simulink model "commhdlQPSKTxRx"  (R2025b)
settings: Solver=FixedStepDiscrete  StartTime=0.0  StopTime=stopTime  RelTol=1e-3
PostLoadFcn:
  | hScopeConfig = get_param([gcs '/Receiver/QPSK Rx/Frequency and Time Synchronizer/Symbol Synchronizer/No HDL/QPSK Receiver Eye Diagram'],'ScopeConfiguration');
  | 
  | hScopeConfig.OpenAtSimulationStart = false;
  | hScopeConfig.Visible = false;
  | SamplesPerSymbol = 4;
  | %UpsamplesRx = 1;
  | clear hScopeConfig
InitFcn:
  | commhdlQPSKTxRxModelInit;
  | % Rate bridge: ADRV9002/Jupiter radio runs at 15.36 MHz = 2x the 7.68 MHz
  | % (4 samples/symbol @ Rsym=1.92 MHz) the QPSK Rx requires. The deployed
  | % Receiver must downsample the ADC stream by 2. UpsamplesRx=1 fed the QPSK
  | % Rx 8 sps (2x-upsampled) and broke symbol sync / the loopback bit check.
  | UpsamplesRx = 1;   %% T8 RATE FIX: rail 15.36e6 == ADC bus rate,
  | %% no ingress decimation (was 2 when the rail sat on the 7.68e6 rung)
  | UpsamplesTx = 1;
  | clear simTimingOffset;
StopFcn:
  | if exist('simTimingOffset','var')
  |   disp('Simulation completed');
  |   %QPSKTxRxVerification;
  | end
undefined symbols (not defined in the file or in its folder): Add, Config, fsym, randsrc, RandStream, Rsym, Shift
libraries: hdlsllib x76, simulink x21, dspsigops x19, dsphdlfiltering2 x3, dsphdlsigops2 x2, dsphdlmathfun2 x2, commdigbbndpm3 x2, commchan3 x1, commrflib2 x1
(part 2 of 4)

== system commhdlQPSKTxRx/Transmitter/QPSK Tx/HDL Data Scrambler ==
  note: HDL Data Scrambler
      | Polynomial: x^7+x^4+1
      | Initial state: [1 0 1 1 1 0 1]
  dataIn : Inport
  startIn : Inport  Port=2
  endIn : Inport  Port=3
  validIn : Inport  Port=4
  BIT_XOR : Logic  Operator=XOR  IconShape=distinctive  AllPortsSameDT=off  OutDataTypeStr=boolean
  BIT_XOR2 : Logic  Operator=XOR  IconShape=distinctive  AllPortsSameDT=off  OutDataTypeStr=boolean
  Delay{,1,3..4} (4 alike) : Delay  DelayLength=1
  EnableScrambling : Constant  Value=true  SampleTime=-1
  Logical Operator : Logic  IconShape=distinctive  AllPortsSameDT=off  OutDataTypeStr=boolean
  Switch : Switch  Criteria=u2 > Threshold  SaturateOnIntegerOverflow=off  InputSameDT=off
  Unit Delay Enabled Resettable Synchronous{,2..3,5,7} (5 alike) : hdlsllib/Discrete/Unit Delay Enabled Resettable Synchronous  InitialCondition=1  SampleTime=-1
  Unit Delay Enabled Resettable Synchronous1 : hdlsllib/Discrete/Unit Delay Enabled Resettable Synchronous  InitialCondition=0  SampleTime=-1
  Unit Delay Enabled Resettable Synchronous4 : hdlsllib/Discrete/Unit Delay Enabled Resettable Synchronous  InitialCondition=0  SampleTime=-1
  Unit Delay Enabled Resettable Synchronous6 : hdlsllib/Discrete/Unit Delay Enabled Resettable Synchronous  InitialCondition=0.0  SampleTime=-1
  dataOut : Outport  InitialOutput=0
  validOut : Outport  Port=2  InitialOutput=0
  wires:
  Delay4/1 -> validOut/1
  Delay3/1 -> dataOut/1
  endIn/1 -> Unit Delay Enabled Resettable Synchronous4/3
  Logical Operator/1 -> BIT_XOR2/2
  Unit Delay Enabled Resettable Synchronous4/1 -> Logical Operator/1
  Delay1/1 -> Unit Delay Enabled Resettable Synchronous6/2, Unit Delay Enabled Resettable Synchronous2/2, Unit Delay Enabled Resettable Synchronous1/2, Unit Delay Enabled Resettable Synchronous/2, Delay4/1, Unit Delay Enabled Resettable Synchronous3/2, Unit Delay Enabled Resettable Synchronous5/2, Unit Delay Enabled Resettable Synchronous7/2
  Delay/1 -> Switch/3, BIT_XOR2/1
  startIn/1 -> Unit Delay Enabled Resettable Synchronous4/1, Unit Delay Enabled Resettable Synchronous4/2, Unit Delay Enabled Resettable Synchronous6/3, Unit Delay Enabled Resettable Synchronous5/3, Unit Delay Enabled Resettable Synchronous1/3, Unit Delay Enabled Resettable Synchronous/3, Unit Delay Enabled Resettable Synchronous2/3, Unit Delay Enabled Resettable Synchronous3/3, Unit Delay Enabled Resettable Synchronous7/3
  dataIn/1 -> Delay/1
  validIn/1 -> Delay1/1
  BIT_XOR/1 -> Unit Delay Enabled Resettable Synchronous/1, Logical Operator/2
  Unit Delay Enabled Resettable Synchronous1/1 -> Unit Delay Enabled Resettable Synchronous2/1
  Unit Delay Enabled Resettable Synchronous2/1 -> Unit Delay Enabled Resettable Synchronous3/1
  Unit Delay Enabled Resettable Synchronous/1 -> Unit Delay Enabled Resettable Synchronous1/1
  Unit Delay Enabled Resettable Synchronous3/1 -> BIT_XOR/2, Unit Delay Enabled Resettable Synchronous5/1
  Unit Delay Enabled Resettable Synchronous5/1 -> Unit Delay Enabled Resettable Synchronous6/1
  Unit Delay Enabled Resettable Synchronous6/1 -> Unit Delay Enabled Resettable Synchronous7/1
  Unit Delay Enabled Resettable Synchronous7/1 -> BIT_XOR/1
  Switch/1 -> Delay3/1
  EnableScrambling/1 -> Switch/2
  BIT_XOR2/1 -> Switch/1

== system commhdlQPSKTxRx/Transmitter/QPSK Tx/QPSK Modulator ==
  dataIn : Inport
  validIn : Inport  Port=2
  Compare To Constant : simulink/Logic and Bit Operations/Compare To Constant  relop===  const=0  OutDataTypeStr=boolean
  Compare To Constant1 : simulink/Logic and Bit Operations/Compare To Constant  relop===  const=1  OutDataTypeStr=boolean
  Delay{,1..5,11..12} (8 alike) : Delay  DelayLength=1
  HDL Counter : hdlsllib/Sources/HDL Counter  CountType=Count limited  CountInit=0  CountStep=1  CountMax=1  CountFromType=Initial value  CountFrom=0  CountResetPort=off  CountLoadPort=off  CountEnbPort=on  CountDirPort=off  CountHitOutputPort=off  CountDataType=Unsigned  CountWordLen=1  CountFracLen=0  CountSampTime=1
  Logical Operator : Logic  IconShape=distinctive  AllPortsSameDT=off  OutDataTypeStr=boolean
  Logical Operator1 : Logic  IconShape=distinctive  AllPortsSameDT=off  OutDataTypeStr=boolean
  Mux : Mux  Inputs=2
  Null : Constant  Value=complex(0,0)  OutDataTypeStr=fixdt(1,16,15)  SampleTime=1/(Rsym*SamplesPerSymbol)
  QPSK Modulator Baseband : commdigbbndpm3/QPSK Modulator Baseband  InType=Bit  Enc=Gray  Ph=pi/4  outDtype=Fixed-point  outWordLen=16  outUDDataType=sfix(16)  outFracLenMode=User-defined  outFracLen=15  outDataTypeStr=fixdt(1,16,15)  outLastDataTypeStr=fixdt(1,16,15)
  Switch3 : Switch  Threshold=1  SaturateOnIntegerOverflow=off  InputSameDT=off
  Unit Delay Enabled Synchronous : hdlsllib/Discrete/Unit Delay Enabled Synchronous  InitialCondition=0.0  SampleTime=-1
  dataOut : Outport
  validOut : Outport  Port=2
  wires:
  dataIn/1 -> Delay/1
  validIn/1 -> Delay1/1
  HDL Counter/1 -> Compare To Constant/1, Compare To Constant1/1
  QPSK Modulator Baseband/1 -> Delay11/1
  Logical Operator1/1 -> Delay5/1
  Switch3/1 -> Delay2/1
  Null/1 -> Switch3/3
  Delay/1 -> Mux/2, Unit Delay Enabled Synchronous/1
  Delay2/1 -> dataOut/1
  Delay3/1 -> validOut/1
  Delay1/1 -> Logical Operator1/2, Logical Operator/1, HDL Counter/1
  Compare To Constant/1 -> Logical Operator/2
  Compare To Constant1/1 -> Logical Operator1/1
  Delay11/1 -> Switch3/1
  Delay12/1 -> Switch3/2, Delay3/1
  Logical Operator/1 -> Unit Delay Enabled Synchronous/2
  Unit Delay Enabled Synchronous/1 -> Mux/1
  Mux/1 -> Delay4/1
  Delay4/1 -> QPSK Modulator Baseband/1
  Delay5/1 -> Delay12/1

== system commhdlQPSKTxRx/Transmitter/QPSK Tx/RRC Transmit Filter ==
  dataIn : Inport
  validIn : Inport  Port=2
  Data Type Conversion : DataTypeConversion  OutDataTypeStr=fixdt(1,17,16)  SaturateOnIntegerOverflow=off  RndMeth=Floor
  Data Type Conversion1 : DataTypeConversion  OutDataTypeStr=fixdt(1,16,14)  SaturateOnIntegerOverflow=off  RndMeth=Floor
  Delay1 : Delay  DelayLength=1
  Delay2 : Delay  DelayLength=1
  Delay3 : Delay  DelayLength=1
  RRC Filter : dsphdlfiltering2/Discrete FIR Filter  NumeratorSource=Property  Numerator=RRCCoef  NumeratorPrototype=[]  FilterStructure=Direct form systolic  SerializationOption=Minimum number of cycles between valid input samples  NumCycles=2  NumberOfMultipliers=2  SimulateUsing=Code generation  roundingMode=Floor  overflowMode=off  CoefficientsDataTypeStr=Inherit: Same word length as input  OutputDataTypeStr=Inherit: Same word length as input  ResetInputPort=off  HDLGlobalReset=off  CoeffMultiplier=Multiplier  UseMultForPow2Coeff=on  FrameInputSymmOptim=off
  Unit Delay Enabled Synchronous1 : hdlsllib/Discrete/Unit Delay Enabled Synchronous  InitialCondition=0  SampleTime=-1
  dataOut : Outport
  validOut : Outport  Port=2
  wires:
  dataIn/1 -> Data Type Conversion/1
  RRC Filter/1 -> Data Type Conversion1/1
  RRC Filter/2 -> Delay2/1
  Delay1/1 -> dataOut/1
  Delay2/1 -> validOut/1
  Data Type Conversion/1 -> Delay3/1
  Unit Delay Enabled Synchronous1/1 -> RRC Filter/2
  Data Type Conversion1/1 -> Delay1/1
  validIn/1 -> Unit Delay Enabled Synchronous1/2, Unit Delay Enabled Synchronous1/1
  Delay3/1 -> RRC Filter/1

== system commhdlQPSKTxRx/Receiver/QPSK Rx/Automatic Gain Control/Error Detector ==
  dataIn : Inport
  Add1 : Sum  Inputs=+-
  Conj : Math  Operator=conj
  Data Type Duplicate : DataTypeDuplicate
  Delay{,1..3} (4 alike) : Delay
  Product : Product
  Ref : Constant  Value=Ref  OutDataTypeStr=Inherit: Inherit via back propagation  SampleTime=-1
  err : Outport
  wires:
  Delay3/1 -> err/1
  Delay2/1 -> Add1/2
  Delay1/1 -> Product/1
  Delay/1 -> Product/2
  Ref/1 -> Data Type Duplicate/1, Add1/1
  Conj/1 -> Delay/1
  Product/1 -> Delay2/1
  dataIn/1 -> Conj/1, Data Type Duplicate/2, Delay1/1
  Add1/1 -> Delay3/1

== system commhdlQPSKTxRx/Receiver/QPSK Rx/Automatic Gain Control/Loop Filter ==
  note: Fixed point precision loss warnings
      | are supressed in Mask Init Callback
  err : Inport
  Add : Sum  Inputs=|++  OutDataTypeStr=Inherit: Same as first input
  Delay1 : Delay  DelayLength=1
  Delay2 : Delay
  Delay3 : Delay
  Gain1 : Gain  Gain=LFG  OutDataTypeStr=fixdt(1,34,28)
      mask init:
      | Simulink.suppressDiagnostic(gcb, 'SimulinkFixedPoint:util:fxpParameterPrecisionLoss');
  gain : Outport
  wires:
  Delay3/1 -> Gain1/1
  Delay2/1 -> Add/1
  Gain1/1 -> Delay2/1
  Add/1 -> Delay1/1
  Delay1/1 -> Add/2, gain/1
  err/1 -> Delay3/1

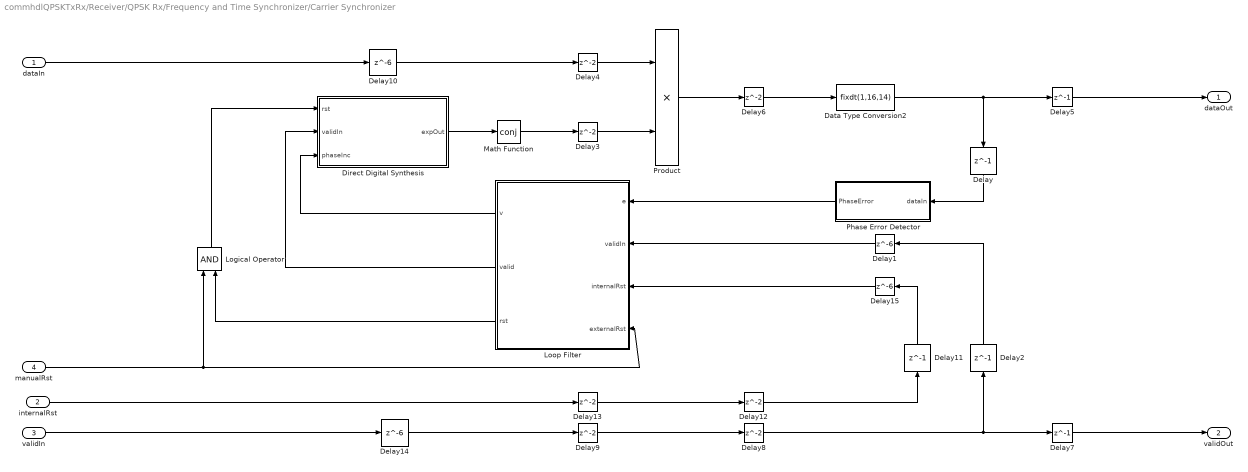
== system commhdlQPSKTxRx/Receiver/QPSK Rx/Frequency and Time Synchronizer/Carrier Synchronizer ==
  dataIn : Inport
  internalRst : Inport  Port=2
  validIn : Inport  Port=3
  manualRst : Inport  Port=4
  Data Type Conversion2 : DataTypeConversion  OutDataTypeStr=fixdt(1,16,14)  SaturateOnIntegerOverflow=off  RndMeth=Floor
  Delay{,2,5,7,11} (5 alike) : Delay  DelayLength=1
  Delay{1,10,14..15} (4 alike) : Delay  DelayLength=6
  Delay{3..4,6,8..9,12..13} (7 alike) : Delay
  Direct Digital Synthesis : Subsystem
  Logical Operator : Logic  AllPortsSameDT=off  OutDataTypeStr=boolean
  Loop Filter : Subsystem
  Math Function : Math  Operator=conj  SignedPower=on  RndMeth=Zero
  Phase Error Detector : Subsystem
  Product : Product
  dataOut : Outport
  validOut : Outport  Port=2
  wires:
  Delay/1 -> Phase Error Detector/1(dataIn)
  Math Function/1 -> Delay3/1
  Data Type Conversion2/1 -> Delay5/1, Delay/1
  Delay3/1 -> Product/2
  Product/1 -> Delay6/1
  Delay8/1 -> Delay2/1, Delay7/1
  Delay9/1 -> Delay8/1
  Delay4/1 -> Product/1
  Delay6/1 -> Data Type Conversion2/1
  Direct Digital Synthesis/1(expOut) -> Math Function/1
  Loop Filter/1(v) -> Direct Digital Synthesis/3(phaseInc)
  Phase Error Detector/1(PhaseError) -> Loop Filter/1(e)
  Delay2/1 -> Delay1/1
  Delay1/1 -> Loop Filter/2(validIn)
  Delay10/1 -> Delay4/1
  Delay11/1 -> Delay15/1
  Delay12/1 -> Delay11/1
  Delay13/1 -> Delay12/1
  Loop Filter/2(valid) -> Direct Digital Synthesis/2(validIn)
  Delay5/1 -> dataOut/1
  Delay7/1 -> validOut/1
  dataIn/1 -> Delay10/1
  internalRst/1 -> Delay13/1
  validIn/1 -> Delay14/1
  Delay14/1 -> Delay9/1
  manualRst/1 -> Logical Operator/1, Loop Filter/4(externalRst)
  Delay15/1 -> Loop Filter/3(internalRst)
  Loop Filter/3(rst) -> Logical Operator/2
  Logical Operator/1 -> Direct Digital Synthesis/1(rst)

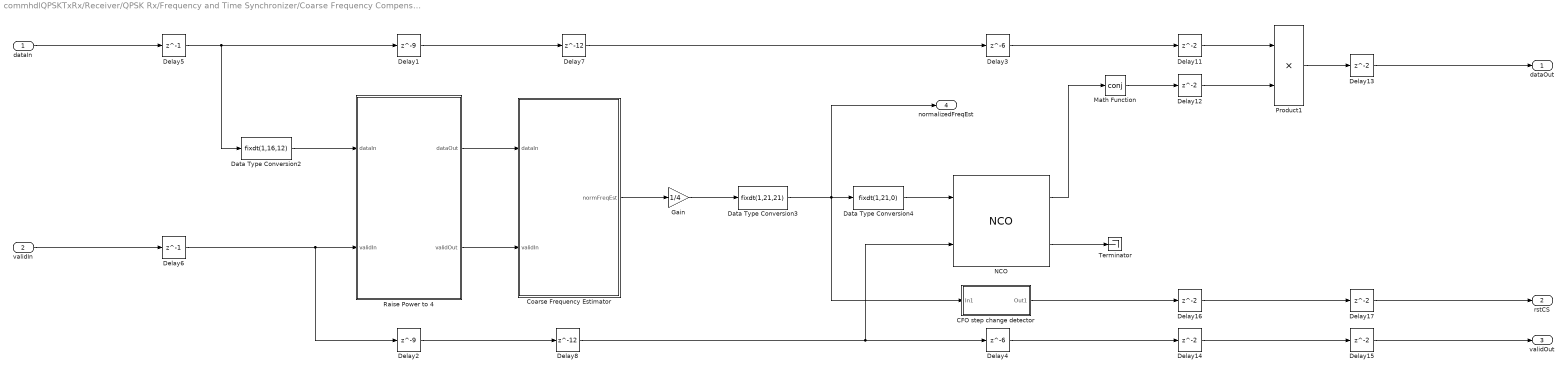
== system commhdlQPSKTxRx/Receiver/QPSK Rx/Frequency and Time Synchronizer/Coarse Frequency Compensator ==
  dataIn : Inport
  validIn : Inport  Port=2
  CFO step change detector : Subsystem
  Coarse Frequency Estimator : Subsystem
  Data Type Conversion2 : DataTypeConversion  OutDataTypeStr=fixdt(1,16,12)  SaturateOnIntegerOverflow=off  RndMeth=Floor
  Data Type Conversion3 : DataTypeConversion  OutDataTypeStr=fixdt(1,21,21)  SaturateOnIntegerOverflow=off  RndMeth=Floor
  Data Type Conversion4 : DataTypeConversion  OutDataTypeStr=fixdt(1,21,0)  ConvertRealWorld=Stored Integer (SI)  SaturateOnIntegerOverflow=off  RndMeth=Floor
  Delay1 : Delay  DelayLength=9
  Delay{11..17} (7 alike) : Delay
  Delay2 : Delay  DelayLength=9
  Delay3 : Delay  DelayLength=6
  Delay4 : Delay  DelayLength=6
  Delay5 : Delay  DelayLength=1
  Delay6 : Delay  DelayLength=1
  Delay7 : Delay  DelayLength=12
  Delay8 : Delay  DelayLength=12
  Gain : Gain  Gain=1/4  ParamDataTypeStr=fixdt(0,2,2)  OutDataTypeStr=Inherit: Same as input
  Math Function : Math  Operator=conj
  NCO : dsphdlsigops2/NCO  PhaseIncrementSource=Input port  PhaseIncrement=100  PhaseOffsetSource=Property  PhaseOffset=0  DitherSource=None  NumDitherBits=4  SamplesPerFrame=1  LUTCompress=off  ResetAction=off  Waveform=Complex exponential  PhasePort=off  SimulateUsing=Code generation  AccumulatorWL=21  PhaseQuantization=on  NumQuantizerAccumulatorBits=14  OutputDataType=Binary point scaling  OutputWL=16  OutputFL=14
  Product1 : Product  OutDataTypeStr=Inherit: Same as first input
  Raise Power to 4 : Subsystem
  Terminator : Terminator
  dataOut : Outport
  rstCS : Outport  Port=2
  validOut : Outport  Port=3
  normalizedFreqEst : Outport  Port=4
  wires:
  Delay14/1 -> Delay15/1
  Delay11/1 -> Product1/1
  Delay6/1 -> Raise Power to 4/2(validIn), Delay2/1
  Delay5/1 -> Delay1/1, Data Type Conversion2/1
  Data Type Conversion4/1 -> NCO/1
  Delay4/1 -> Delay14/1
  Delay3/1 -> Delay11/1
  Delay2/1 -> Delay8/1
  Delay1/1 -> Delay7/1
  NCO/2 -> Terminator/1
  NCO/1 -> Math Function/1
  Product1/1 -> Delay13/1
  Raise Power to 4/2(validOut) -> Coarse Frequency Estimator/2(validIn)
  Math Function/1 -> Delay12/1
  Raise Power to 4/1(dataOut) -> Coarse Frequency Estimator/1(dataIn)
  Delay12/1 -> Product1/2
  Coarse Frequency Estimator/1(normFreqEst) -> Gain/1
  Data Type Conversion2/1 -> Raise Power to 4/1(dataIn)
  Delay16/1 -> Delay17/1
  CFO step change detector/1(Out1) -> Delay16/1
  Gain/1 -> Data Type Conversion3/1
  Delay13/1 -> dataOut/1
  dataIn/1 -> Delay5/1
  validIn/1 -> Delay6/1
  Delay17/1 -> rstCS/1
  Data Type Conversion3/1 -> normalizedFreqEst/1, CFO step change detector/1(In1), Data Type Conversion4/1
  Delay15/1 -> validOut/1
  Delay7/1 -> Delay3/1
  Delay8/1 -> NCO/2, Delay4/1

== system commhdlQPSKTxRx/Receiver/QPSK Rx/Frequency and Time Synchronizer/No HDL ==
  In1 : Inport
  In2 : Inport  Port=2
  In3 : Inport  Port=3
  In4 : Inport  Port=4
  Data Type Conversion : DataTypeConversion  OutDataTypeStr=double  SaturateOnIntegerOverflow=off  RndMeth=Floor
  Data Type Conversion1 : DataTypeConversion  OutDataTypeStr=double  SaturateOnIntegerOverflow=off  RndMeth=Floor
  QPSK Receiver Constellations 2 : ConstellationDiagram  NumInputPorts=2  WindowPosition=[67.000000,180.000000,973.000000,678.000000,]  Visible=on  ScopeFrameLocation=window  SymbolsToDisplaySource=Property  SymbolsToDisplay=10000  ReferenceConstellation="{[0.70711+0.70711i        -0.70711+0.70711i        -0.70711-0.70711i         0.70711-0.70711i],[0.70711+0.70711i        -0.70711+0.70711i        -0.70711-0.70711i         0.70711-0.70711i]}"  ReferenceMarker={''+'',''+''}  ReferenceColor={[1 0 0],[1 0 0]}  XLimits=[-1.3581 1.3569]  YLimits=[-1.3581 1.3569]  AxesLimits=[-1.3581 1.3569]  ShowLegend=on  DefaultConfigurationName=comm.scopes.ConstellationDiagramBlockCfg
      settings: OpenAtSimulationStart=off
  Subsystem : Subsystem
  Unit Delay Enabled Synchronous : hdlsllib/Discrete/Unit Delay Enabled Synchronous  InitialCondition=0.0  SampleTime=-1
  Unit Delay Enabled Synchronous1 : hdlsllib/Discrete/Unit Delay Enabled Synchronous  InitialCondition=0.0  SampleTime=-1
  wires:
  In4/1 -> Unit Delay Enabled Synchronous1/2, Subsystem/Enable
  Data Type Conversion/1 -> Unit Delay Enabled Synchronous1/1, Subsystem/1(In1)
  Unit Delay Enabled Synchronous1/1 -> QPSK Receiver Constellations 2/2  "After Carrier Synchronization"
  In2/1 -> Unit Delay Enabled Synchronous/2
  In1/1 -> Data Type Conversion1/1
  Data Type Conversion1/1 -> Unit Delay Enabled Synchronous/1
  Unit Delay Enabled Synchronous/1 -> QPSK Receiver Constellations 2/1  "After Symbol Synchronization"
  In3/1 -> Data Type Conversion/1

== system commhdlQPSKTxRx/Receiver/QPSK Rx/Frequency and Time Synchronizer/Packet Controller ==
  dataIn : Inport
  syncPulse : Inport  Port=2
  validIn : Inport  Port=3
  Delay : Delay  DelayLength=4
  Delay1 : Delay  DelayLength=4
  Delay2 : Delay  DelayLength=4
  End Generator : Subsystem
  Logical Operator : Logic  IconShape=distinctive  AllPortsSameDT=off  OutDataTypeStr=boolean
  MATLAB Function : MATLAB Function  TreatAsAtomicUnit=on
  Time Scope End Generator : Scope  Commented=on  NumInputPorts=2
      settings: SampleTime=1  ActiveDisplayYMinimum=-0.048155737704917989  ActiveDisplayYMaximum=1.0464480874316939  YLabel=Amplitude  DataLoggingVariableName=ScopeData2
  To File : ToFile  Filename=end_gen.mat  MatrixName=end_gen  SaveFormat=Timeseries
  To File1 : ToFile  Filename=reset  MatrixName=reset  SaveFormat=Timeseries
  sample discard controller : MATLAB Function  TreatAsAtomicUnit=on
  dataOut : Outport
  startOut : Outport  Port=2
  endOut : Outport  Port=3
  validOut : Outport  Port=4
  wires:
  MATLAB Function/1(out) -> Logical Operator/2
  sample discard controller/1(dataOut) -> dataOut/1
  sample discard controller/2(startOut) -> startOut/1
  sample discard controller/3(endOut) -> endOut/1
  sample discard controller/4(validOut) -> validOut/1
  Delay/1 -> sample discard controller/1(dataIn)
  Delay1/1 -> sample discard controller/2(validIn), End Generator/1(validIn)
  Delay2/1 -> sample discard controller/3(startIn)
  dataIn/1 -> Delay/1
  validIn/1 -> MATLAB Function/1(valid), Delay1/1, Logical Operator/1
  Logical Operator/1 -> Delay2/1, To File1/1, Time Scope End Generator/2, End Generator/2(rst)
  syncPulse/1 -> MATLAB Function/2(syncPulse)
  End Generator/1(endOut) -> Time Scope End Generator/1, To File/1, sample discard controller/4(endIn)

== system commhdlQPSKTxRx/Receiver/QPSK Rx/Frequency and Time Synchronizer/Phase Ambiguity Estimation and Correction ==
  dataIn : Inport
  syncPulseIn : Inport  Port=2
  validIn : Inport  Port=3
  Average Estimates : Subsystem
  Delay : Delay  DelayLength=32
  Delay1 : Delay  DelayLength=32
  Delay10 : Delay  DelayLength=15 + 7
  Delay11 : Delay  DelayLength=5
  Delay12 : Delay  DelayLength=5
  Delay13 : Delay  DelayLength=5
  Delay2 : Delay  DelayLength=32
  Delay3 : Delay  DelayLength=8
  Delay4 : Delay  DelayLength=8
  Delay5 : Delay  DelayLength=8
  Delay6 : Delay  DelayLength=1
  Delay7 : Delay  DelayLength=1
  Delay8 : Delay  DelayLength=1
  Delay9 : Delay  DelayLength=10
  Phase Ambiguity Corrector : Subsystem
  Phase Ambiguity Estimator : Subsystem
  dataOut : Outport
  syncPulseOut : Outport  Port=2
  validOut : Outport  Port=3
  wires:
  Delay4/1 -> Delay2/1
  Delay5/1 -> Delay/1
  Delay3/1 -> Delay1/1
  Delay10/1 -> Delay9/1
  Phase Ambiguity Corrector/1(dataOut) -> dataOut/1
  Phase Ambiguity Corrector/2(validOut) -> validOut/1
  Delay9/1 -> syncPulseOut/1
  Delay8/1 -> Phase Ambiguity Corrector/1(dataIn)
  Average Estimates/1(avgEst) -> Phase Ambiguity Corrector/2(estimate)
  Delay7/1 -> Phase Ambiguity Corrector/3(validIn)
  Delay6/1 -> Delay10/1
  dataIn/1 -> Delay5/1
  validIn/1 -> Delay4/1
  Delay13/1 -> Delay8/1
  Phase Ambiguity Estimator/1(endOut) -> Average Estimates/1(endIn)
  Phase Ambiguity Estimator/3(validOut) -> Average Estimates/3(validIn)
  Delay12/1 -> Delay7/1
  Delay11/1 -> Delay6/1
  Phase Ambiguity Estimator/2(estOut) -> Average Estimates/2(estin)
  Delay/1 -> Delay13/1, Phase Ambiguity Estimator/1(dataIn)
  syncPulseIn/1 -> Phase Ambiguity Estimator/2(syncPulse), Delay3/1
  Delay2/1 -> Phase Ambiguity Estimator/3(validIn), Delay12/1
  Delay1/1 -> Delay11/1

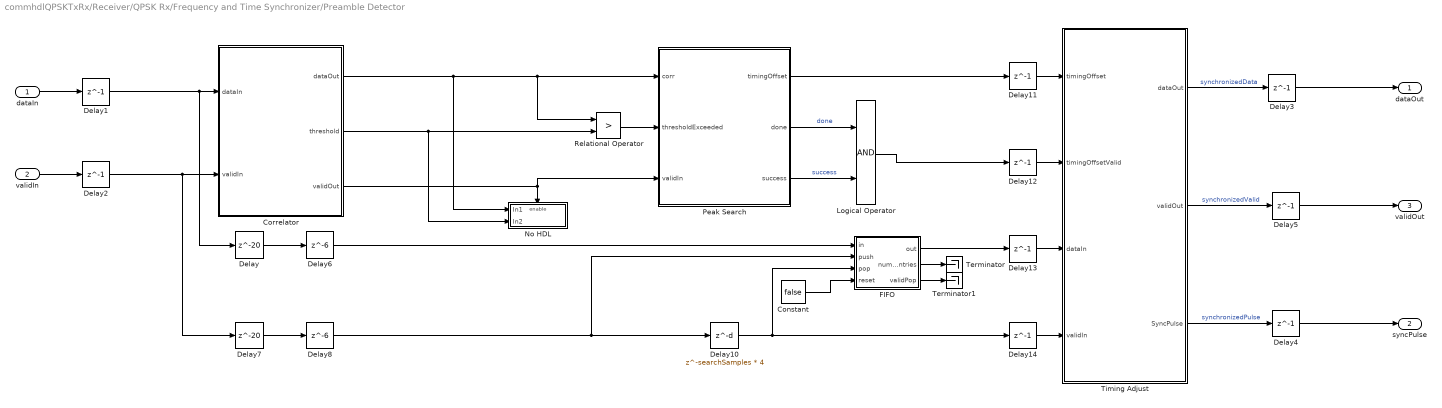
== system commhdlQPSKTxRx/Receiver/QPSK Rx/Frequency and Time Synchronizer/Preamble Detector ==
  dataIn : Inport
  validIn : Inport  Port=2
  Constant : Constant  Value=false  SampleTime=-1
  Correlator : Subsystem
  Delay : Delay  DelayLength=20
  Delay{1..5,11..14} (9 alike) : Delay  DelayLength=1
  Delay10 : Delay  DelayLength=searchSamples * 4
  Delay6 : Delay  DelayLength=6
  Delay7 : Delay  DelayLength=20
  Delay8 : Delay  DelayLength=6
  FIFO : Subsystem  mask{fifoSize=searchSamples, pushFullDiag=Error, popEmptyDiag=Error}
      mask prompts: fifoSize "FIFO size:"; pushFullDiag "Push full FIFO:"; popEmptyDiag "Pop empty FIFO:"
      mask TypeOptions pushFullDiag: Ignore | Warning | Error
      mask TypeOptions popEmptyDiag: Ignore | Warning | Error
  Logical Operator : Logic  AllPortsSameDT=off  OutDataTypeStr=boolean
  No HDL : Subsystem
  Peak Search : Subsystem  VariantControl=new  mask{samplesPerFrame=searchSamples}
      mask prompts: samplesPerFrame "Number of samples to search:"
      mask init:
      | samplesPerFrame1x            = samplesPerFrame;
      |     searchDuration               = samplesPerFrame1x;
  Relational Operator : RelationalOperator  Operator=>  OutDataTypeStr=boolean  InputSameDT=off
  Terminator : Terminator
  Terminator1 : Terminator
  Timing Adjust : Subsystem
  dataOut : Outport
  syncPulse : Outport  Port=2
  validOut : Outport  Port=3
  wires:
  Delay/1 -> Delay6/1
  validIn/1 -> Delay2/1
  dataIn/1 -> Delay1/1
  Relational Operator/1 -> Peak Search/2(thresholdExceeded)
  Peak Search/3(success) -> Logical Operator/2  "success"
  Peak Search/2(done) -> Logical Operator/1  "done"
  Delay7/1 -> Delay8/1
  Timing Adjust/1(dataOut) -> Delay3/1  "synchronizedData"
  Timing Adjust/3(SyncPulse) -> Delay4/1  "synchronizedPulse"
  Timing Adjust/2(validOut) -> Delay5/1  "synchronizedValid"
  Delay3/1 -> dataOut/1
  Delay5/1 -> validOut/1
  Delay4/1 -> syncPulse/1
  Peak Search/1(timingOffset) -> Delay11/1
  Logical Operator/1 -> Delay12/1
  Delay10/1 -> FIFO/3(pop), Delay14/1
  Correlator/3(validOut) -> Peak Search/3(validIn), No HDL/Enable
  Correlator/2(threshold) -> Relational Operator/2, No HDL/2(In2)
  Correlator/1(dataOut) -> Relational Operator/1, Peak Search/1(corr), No HDL/1(In1)
  Delay8/1 -> FIFO/2(push), Delay10/1
  Delay1/1 -> Delay/1, Correlator/1(dataIn)
  Delay2/1 -> Delay7/1, Correlator/2(validIn)
  Delay11/1 -> Timing Adjust/1(timingOffset)
  Delay12/1 -> Timing Adjust/2(timingOffsetValid)
  Delay13/1 -> Timing Adjust/3(dataIn)
  Delay14/1 -> Timing Adjust/4(validIn)
  FIFO/2(numEntries) -> Terminator/1
  Constant/1 -> FIFO/4(reset)
  FIFO/3(validPop) -> Terminator1/1
  Delay6/1 -> FIFO/1(in)
  FIFO/1(out) -> Delay13/1

== system commhdlQPSKTxRx/Receiver/QPSK Rx/Frequency and Time Synchronizer/Symbol Synchronizer ==
  dataIn : Inport
  validIn : Inport  Port=2
  Data Type Conversion4 : DataTypeConversion  OutDataTypeStr=fixdt(1,16,14)  SaturateOnIntegerOverflow=off  RndMeth=Floor
  Delay{1..4,6,8..9} (7 alike) : Delay  DelayLength=1
  Delay5 : Delay  DelayLength=12
  Delay7 : Delay  DelayLength=12
  Gardner TED : Subsystem
  Integer Delay{1..4} (4 alike) : Delay  DelayLength=1
  Interpolation Control : MATLAB Function
  Interpolation Filter : Subsystem
  Loop Filter : Subsystem
  No HDL : Subsystem
  Rate Handle : Subsystem
  dataOut : Outport
  validOut : Outport  Port=2
  wires:
  Loop Filter/1(v) -> Delay4/1
  Gardner TED/1(e) -> Delay3/1
  Interpolation Control/2(Underflow) -> Integer Delay3/1
  Integer Delay4/1 -> Interpolation Filter/2(mu)
  dataIn/1 -> No HDL/1(data), Integer Delay1/1
  Integer Delay3/1 -> Delay5/1
  Delay3/1 -> Loop Filter/1(e)
  Delay4/1 -> Interpolation Control/1(Delta)
  Data Type Conversion4/1 -> Rate Handle/1(dataIn)
  Delay1/1 -> Data Type Conversion4/1
  Delay6/1 -> Rate Handle/3(validIn)
  Delay7/1 -> Delay6/1
  validIn/1 -> No HDL/2(valid), Integer Delay2/1
  Rate Handle/2(validOut) -> validOut/1
  Rate Handle/1(dataOut) -> dataOut/1
  Interpolation Filter/1(interpolant) -> Delay8/1, Delay1/1
  Interpolation Control/1(mu) -> Integer Delay4/1
  Delay2/1 -> Rate Handle/2(strobe)
  Delay5/1 -> Delay9/1, Delay2/1
  Integer Delay1/1 -> Interpolation Filter/1(In)
  Integer Delay2/1 -> Delay7/1
  Delay8/1 -> Gardner TED/1(data)
  Delay9/1 -> Gardner TED/2(strobe)

== system commhdlQPSKTxRx/Receiver/QPSK Rx/QPSK Demodulator/Serializer ==
  u : Inport
  In2 : Inport  Port=2
  Delay1 : Delay  DelayLength=1
  Delay4 : Delay  DelayLength=1
  Demux : Demux  Outputs=2
  HDL Counter : hdlsllib/Sources/HDL Counter  CountType=Count limited  CountInit=0  CountStep=1  CountMax=1  CountFromType=Initial value  CountFrom=0  CountResetPort=off  CountLoadPort=off  CountEnbPort=on  CountDirPort=off  CountHitOutputPort=off  CountDataType=Unsigned  CountWordLen=1  CountFracLen=0  CountSampTime=1
  Logical Operator : Logic  Operator=OR  AllPortsSameDT=off  OutDataTypeStr=boolean
  Multiport Switch : MultiPortSwitch  DataPortOrder=Zero-based contiguous  Inputs=2  zeroidx=on  SaturateOnIntegerOverflow=off  InputSameDT=off
  Unit Delay Enabled Synchronous : hdlsllib/Discrete/Unit Delay Enabled Synchronous  InitialCondition=0.0  SampleTime=-1
  Out1 : Outport
  Out2 : Outport  Port=2
  wires:
  Demux/2 -> Multiport Switch/3
  Logical Operator/1 -> Out2/1, HDL Counter/1
  In2/1 -> Unit Delay Enabled Synchronous/2, Delay1/1
  HDL Counter/1 -> Multiport Switch/1
  Delay4/1 -> Logical Operator/2
  u/1 -> Unit Delay Enabled Synchronous/1
  Multiport Switch/1 -> Out1/1
  Demux/1 -> Multiport Switch/2
  Delay1/1 -> Logical Operator/1, Delay4/1
  Unit Delay Enabled Synchronous/1 -> Demux/1

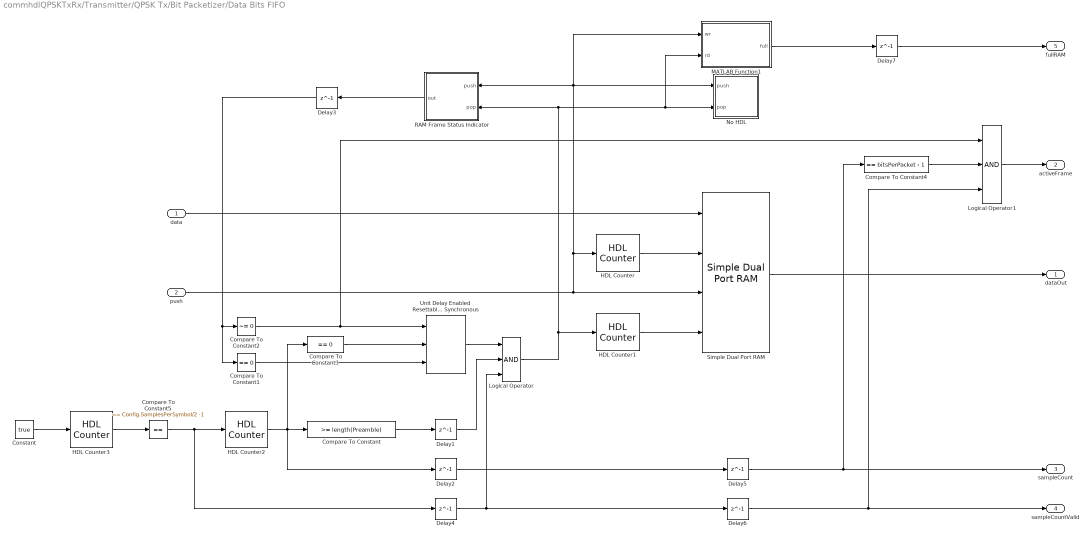
== system commhdlQPSKTxRx/Transmitter/QPSK Tx/Bit Packetizer/Data Bits FIFO ==
  data : Inport
  push : Inport  Port=2
  Compare To Constant : simulink/Logic and Bit Operations/Compare To Constant  relop=>=  const=length(Preamble)  OutDataTypeStr=boolean
  Compare To Constant1 : simulink/Logic and Bit Operations/Compare To Constant  relop===  const=0  OutDataTypeStr=boolean
  Compare To Constant2 : simulink/Logic and Bit Operations/Compare To Constant  relop=~=  const=0  OutDataTypeStr=boolean
  Compare To Constant3 : simulink/Logic and Bit Operations/Compare To Constant  relop===  const=0  OutDataTypeStr=boolean
  Compare To Constant4 : simulink/Logic and Bit Operations/Compare To Constant  relop===  const=bitsPerPacket - 1  OutDataTypeStr=boolean
  Compare To Constant5 : hdlsllib/Logic and Bit Operations/Compare To Constant  relop===  const=Config.SamplesPerSymbol/2 -1  OutDataTypeStr=boolean
  Constant : Constant  Value=true  SampleTime=1/(Rsym*SamplesPerSymbol)
  Delay{1..7} (7 alike) : Delay  DelayLength=1
  HDL Counter : hdlsllib/Sources/HDL Counter  CountType=Count limited  CountInit=0  CountStep=1  CountMax=dataBitsPerPacket*2 - 1  CountFromType=Initial value  CountFrom=0  CountResetPort=off  CountLoadPort=off  CountEnbPort=on  CountDirPort=off  CountHitOutputPort=off  CountDataType=Unsigned  CountWordLen=nextpow2(dataBitsPerPacket*2 - 1)  CountFracLen=0  CountSampTime=1
  HDL Counter1 : hdlsllib/Sources/HDL Counter  CountType=Count limited  CountInit=0  CountStep=1  CountMax=dataBitsPerPacket*2 - 1  CountFromType=Initial value  CountFrom=0  CountResetPort=off  CountLoadPort=off  CountEnbPort=on  CountDirPort=off  CountHitOutputPort=off  CountDataType=Unsigned  CountWordLen=nextpow2(dataBitsPerPacket*2 - 1)  CountFracLen=0  CountSampTime=1
  HDL Counter2 : hdlsllib/Sources/HDL Counter  CountType=Count limited  CountInit=0  CountStep=1  CountMax=bitsPerPacket - 1  CountFromType=Initial value  CountFrom=0  CountResetPort=off  CountLoadPort=off  CountEnbPort=on  CountDirPort=off  CountHitOutputPort=off  CountDataType=Unsigned  CountWordLen=nextpow2(bitsPerPacket)  CountFracLen=0  CountSampTime=1
  HDL Counter3 : hdlsllib/Sources/HDL Counter  CountType=Count limited  CountInit=0  CountStep=1  CountMax=Config.SamplesPerSymbol/2 -1  CountFromType=Initial value  CountFrom=0  CountResetPort=off  CountLoadPort=off  CountEnbPort=on  CountDirPort=off  CountHitOutputPort=off  CountDataType=Unsigned  CountWordLen=nextpow2(Config.SamplesPerSymbol/2)  CountFracLen=0  CountSampTime=1
  Logical Operator : Logic  Inputs=3  AllPortsSameDT=off  OutDataTypeStr=boolean
  Logical Operator1 : Logic  Inputs=3  AllPortsSameDT=off  OutDataTypeStr=boolean
  MATLAB Function1 : MATLAB Function  TreatAsAtomicUnit=on
  No HDL : Subsystem
  RAM Frame Status Indicator : MATLAB Function  TreatAsAtomicUnit=on
  Simple Dual Port RAM : hdlsllib/HDL RAMs/Simple Dual Port RAM  ram_size=nextpow2(dataBitsPerPacket*2 - 1)
  Unit Delay Enabled Resettable Synchronous : hdlsllib/Discrete/Unit Delay Enabled Resettable Synchronous  InitialCondition=0.0  SampleTime=-1
  dataOut : Outport
  activeFrame : Outport  Port=2
  sampleCount : Outport  Port=3
  sampleCountValid : Outport  Port=4
  fullRAM : Outport  Port=5
  wires:
  HDL Counter1/1 -> Simple Dual Port RAM/4
  HDL Counter/1 -> Simple Dual Port RAM/2
  data/1 -> Simple Dual Port RAM/1
  Constant/1 -> HDL Counter3/1
  HDL Counter2/1 -> Compare To Constant/1, Delay2/1, Compare To Constant3/1
  Compare To Constant1/1 -> Unit Delay Enabled Resettable Synchronous/3
  RAM Frame Status Indicator/1(out) -> Delay3/1
  Compare To Constant2/1 -> Logical Operator1/1, Unit Delay Enabled Resettable Synchronous/1
  Compare To Constant3/1 -> Unit Delay Enabled Resettable Synchronous/2
  Compare To Constant/1 -> Delay1/1
  Delay1/1 -> Logical Operator/2
  Delay2/1 -> Delay5/1
  Delay3/1 -> Compare To Constant2/1, Compare To Constant1/1
  Simple Dual Port RAM/1 -> dataOut/1
  Delay4/1 -> Logical Operator/3, Delay6/1
  Delay5/1 -> Compare To Constant4/1, sampleCount/1
  Delay6/1 -> Logical Operator1/3, sampleCountValid/1
  Unit Delay Enabled Resettable Synchronous/1 -> Logical Operator/1
  Compare To Constant4/1 -> Logical Operator1/2
  Logical Operator1/1 -> activeFrame/1
  Logical Operator/1 -> RAM Frame Status Indicator/2(pop), MATLAB Function1/2(rd), No HDL/2(pop), HDL Counter1/1
  push/1 -> MATLAB Function1/1(wr), RAM Frame Status Indicator/1(push), No HDL/1(push), HDL Counter/1, Simple Dual Port RAM/3
  MATLAB Function1/1(full) -> Delay7/1
  Delay7/1 -> fullRAM/1
  HDL Counter3/1 -> Compare To Constant5/1
  Compare To Constant5/1 -> HDL Counter2/1, Delay4/1

== system commhdlQPSKTxRx/Transmitter/QPSK Tx/Bit Packetizer/Preamble Bits Generator ==
  activeFrame : Inport
  sampleCount : Inport  Port=2
  sampleCountValid : Inport  Port=3
  Compare To Constant2 : hdlsllib/Logic and Bit Operations/Compare To Constant  relop===  const=bitsPerPacket - 1  OutDataTypeStr=boolean
  Logical Operator3 : Logic  AllPortsSameDT=off  OutDataTypeStr=boolean
  Preamble Bits Store : Subsystem
  Unit Delay Enabled Synchronous : hdlsllib/Discrete/Unit Delay Enabled Synchronous  InitialCondition=0.0  SampleTime=-1
  preambleBits : Outport
  wires:
  sampleCount/1 -> Compare To Constant2/1, Preamble Bits Store/2(sampleCount)
  Logical Operator3/1 -> Unit Delay Enabled Synchronous/2
  Preamble Bits Store/1(preamble) -> preambleBits/1
  Compare To Constant2/1 -> Logical Operator3/1
  Unit Delay Enabled Synchronous/1 -> Preamble Bits Store/1(actualPreamble)
  sampleCountValid/1 -> Logical Operator3/2
  activeFrame/1 -> Unit Delay Enabled Synchronous/1

== system commhdlQPSKTxRx/Receiver/QPSK Rx/Frequency and Time Synchronizer/Carrier Synchronizer/Direct Digital Synthesis ==
  rst : Inport
  validIn : Inport  Port=2
  phaseInc : Inport  Port=3
  Data Type Conversion : DataTypeConversion  OutDataTypeStr=fixdt(1,21,21)  SaturateOnIntegerOverflow=off  RndMeth=Floor
  Data Type Conversion1 : DataTypeConversion  OutDataTypeStr=fixdt(1,21,0)  ConvertRealWorld=Stored Integer (SI)  SaturateOnIntegerOverflow=off  RndMeth=Floor
  Delay : Delay  DelayLength=1
  NCO : dsphdlsigops2/NCO  PhaseIncrementSource=Input port  PhaseIncrement=0  PhaseOffsetSource=Property  PhaseOffset=0  DitherSource=Property  NumDitherBits=11  SamplesPerFrame=1  LUTCompress=off  ResetAction=on  Waveform=Complex exponential  PhasePort=off  SimulateUsing=Code generation  AccumulatorWL=21  PhaseQuantization=on  NumQuantizerAccumulatorBits=14  OutputDataType=Binary point scaling  OutputWL=16  OutputFL=14
  Terminator : Terminator
  expOut : Outport
  wires:
  Data Type Conversion/1 -> Data Type Conversion1/1
  NCO/1 -> expOut/1
  validIn/1 -> NCO/3
  Data Type Conversion1/1 -> NCO/1
  NCO/2 -> Terminator/1
  Delay/1 -> Data Type Conversion/1
  phaseInc/1 -> Delay/1
  rst/1 -> NCO/2

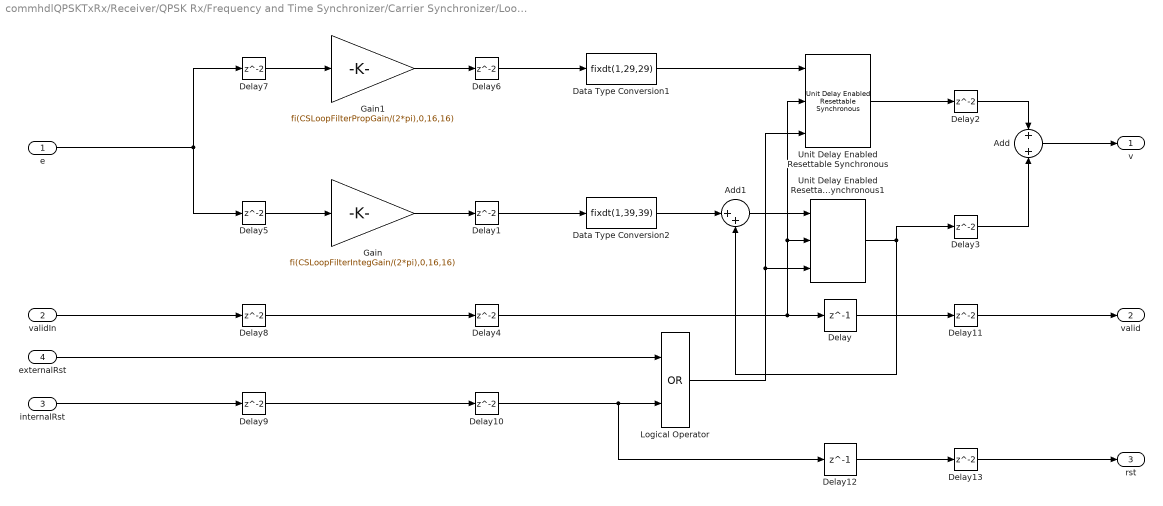
== system commhdlQPSKTxRx/Receiver/QPSK Rx/Frequency and Time Synchronizer/Carrier Synchronizer/Loop Filter ==
  e : Inport
  validIn : Inport  Port=2
  internalRst : Inport  Port=3
  externalRst : Inport  Port=4
  Add : Sum  Inputs=+|+
  Add1 : Sum  Inputs=|++  OutDataTypeStr=Inherit: Same as first input
  Data Type Conversion1 : DataTypeConversion  OutDataTypeStr=fixdt(1,29,29)  SaturateOnIntegerOverflow=off  RndMeth=Floor
  Data Type Conversion2 : DataTypeConversion  OutDataTypeStr=fixdt(1,39,39)  SaturateOnIntegerOverflow=off  RndMeth=Floor
  Delay : Delay  DelayLength=1
  Delay{1..11,13} (12 alike) : Delay
  Delay12 : Delay  DelayLength=1
  Gain : Gain  Gain=fi(CSLoopFilterIntegGain/(2*pi),0,16,16)  ParamDataTypeStr=Inherit: Inherit from 'Gain'
  Gain1 : Gain  Gain=fi(CSLoopFilterPropGain/(2*pi),0,16,16)  ParamDataTypeStr=Inherit: Inherit from 'Gain'
  Logical Operator : Logic  Operator=OR  AllPortsSameDT=off  OutDataTypeStr=boolean
  Unit Delay Enabled Resettable Synchronous : hdlsllib/Discrete/Unit Delay Enabled Resettable Synchronous  InitialCondition=0.0  SampleTime=-1
  Unit Delay Enabled Resettable Synchronous1 : hdlsllib/Discrete/Unit Delay Enabled Resettable Synchronous  InitialCondition=0.0  SampleTime=-1
  v : Outport
  valid : Outport  Port=2
  rst : Outport  Port=3
  wires:
  Delay6/1 -> Data Type Conversion1/1
  Delay5/1 -> Gain/1
  Delay7/1 -> Gain1/1
  Gain/1 -> Delay1/1
  Data Type Conversion2/1 -> Add1/1
  Delay3/1 -> Add/2
  Delay1/1 -> Data Type Conversion2/1
  Gain1/1 -> Delay6/1
  Delay2/1 -> Add/1
  Add/1 -> v/1
  e/1 -> Delay7/1, Delay5/1
  Data Type Conversion1/1 -> Unit Delay Enabled Resettable Synchronous/1
  Add1/1 -> Unit Delay Enabled Resettable Synchronous1/1
  Unit Delay Enabled Resettable Synchronous1/1 -> Delay3/1, Add1/2
  Unit Delay Enabled Resettable Synchronous/1 -> Delay2/1
  Logical Operator/1 -> Unit Delay Enabled Resettable Synchronous/3, Unit Delay Enabled Resettable Synchronous1/3
  validIn/1 -> Delay8/1
  Delay8/1 -> Delay4/1
  externalRst/1 -> Logical Operator/1
  internalRst/1 -> Delay9/1
  Delay9/1 -> Delay10/1
  Delay10/1 -> Delay12/1, Logical Operator/2
  Delay4/1 -> Unit Delay Enabled Resettable Synchronous/2, Unit Delay Enabled Resettable Synchronous1/2, Delay/1
  Delay11/1 -> valid/1
  Delay/1 -> Delay11/1
  Delay12/1 -> Delay13/1
  Delay13/1 -> rst/1

== system commhdlQPSKTxRx/Receiver/QPSK Rx/Frequency and Time Synchronizer/Carrier Synchronizer/Phase Error Detector ==
  dataIn : Inport
  Add : Sum  Inputs=+|-
  Compare To Constant : simulink/Logic and Bit Operations/Compare To Constant  relop=>=  const=0  OutDataTypeStr=boolean
  Compare To Constant1 : simulink/Logic and Bit Operations/Compare To Constant  relop=>=  const=0  OutDataTypeStr=boolean
  Complex to Real-Imag : ComplexToRealImag
  Constant : Constant  OutDataTypeStr=fixdt(1,2,0)  SampleTime=1/(Rsym*SamplesPerSymbol)
  Constant1 : Constant  Value=-1  OutDataTypeStr=fixdt(1,2,0)  SampleTime=1/(Rsym*SamplesPerSymbol)
  Constant2 : Constant  OutDataTypeStr=fixdt(1,2,0)  SampleTime=1/(Rsym*SamplesPerSymbol)
  Constant3 : Constant  Value=-1  OutDataTypeStr=fixdt(1,2,0)  SampleTime=1/(Rsym*SamplesPerSymbol)
  Data Type Conversion3 : DataTypeConversion  OutDataTypeStr=fixdt(1,10+3,10)  SaturateOnIntegerOverflow=off  RndMeth=Floor
  Delay{,1..6} (7 alike) : Delay
  Product : Product
  Product1 : Product
  Switch : Switch  Threshold=1  SaturateOnIntegerOverflow=off  InputSameDT=off
  Switch1 : Switch  Threshold=1  SaturateOnIntegerOverflow=off  InputSameDT=off
  PhaseError : Outport
  wires:
  Complex to Real-Imag/1 -> Delay2/1, Compare To Constant/1
  Compare To Constant1/1 -> Switch1/2
  Constant/1 -> Switch/1
  Constant3/1 -> Switch1/3
  Constant2/1 -> Switch1/1
  Constant1/1 -> Switch/3
  Compare To Constant/1 -> Switch/2
  Add/1 -> Delay6/1
  Switch/1 -> Delay/1
  Product1/1 -> Delay5/1
  Product/1 -> Delay4/1
  Switch1/1 -> Delay3/1
  Complex to Real-Imag/2 -> Delay1/1, Compare To Constant1/1
  dataIn/1 -> Complex to Real-Imag/1
  Delay/1 -> Product/1
  Delay1/1 -> Product/2
  Delay2/1 -> Product1/1
  Delay3/1 -> Product1/2
  Delay4/1 -> Add/1
  Delay5/1 -> Add/2
  Delay6/1 -> Data Type Conversion3/1
  Data Type Conversion3/1 -> PhaseError/1

== system commhdlQPSKTxRx/Receiver/QPSK Rx/Frequency and Time Synchronizer/Coarse Frequency Compensator/CFO step change detector ==
  note: fixed point precision loss warning supressed for this subsystem
  In1 : Inport
  Add : Sum  Inputs=+-
  Compare To Constant : simulink/Logic and Bit Operations/Compare To Constant  relop=>  const=fi(CFOChangeDetectThreshold,1,22,21)  OutDataTypeStr=boolean
  Compare To Constant1 : simulink/Logic and Bit Operations/Compare To Constant  relop=<  const=fi(-CFOChangeDetectThreshold,1,22,21)  OutDataTypeStr=boolean
  Delay : Delay  DelayLength=6
  Delay1 : Delay  DelayLength=1
  Logical Operator : Logic  Operator=OR  AllPortsSameDT=off  OutDataTypeStr=boolean
  Out1 : Outport
  wires:
  In1/1 -> Add/1, Delay1/1
  Delay/1 -> Out1/1
  Delay1/1 -> Add/2
  Add/1 -> Compare To Constant/1, Compare To Constant1/1
  Compare To Constant/1 -> Logical Operator/1
  Logical Operator/1 -> Delay/1
  Compare To Constant1/1 -> Logical Operator/2

== system commhdlQPSKTxRx/Receiver/QPSK Rx/Frequency and Time Synchronizer/Coarse Frequency Compensator/Coarse Frequency Estimator ==
  dataIn : Inport
  validIn : Inport  Port=2
  Delay{1,9..12} (5 alike) : Delay  DelayLength=1
  Delay{2..8} (7 alike) : Delay
  Extract Frequency : Subsystem
  Gain1 : Gain  Gain=1/integAvgLen  ParamDataTypeStr=fixdt(0,nextpow2(integAvgLen),nextpow2(integAvgLen))  OutDataTypeStr=Inherit: Same as input
  Integrator : Subsystem
  Math Function : Math  Operator=conj
  Product : Product
  Unit Delay Enabled Synchronous : hdlsllib/Discrete/Unit Delay Enabled Synchronous  InitialCondition=0.0  SampleTime=-1
  normFreqEst : Outport
  wires:
  Delay8/1 -> Product/2
  Delay7/1 -> Product/1
  Delay6/1 -> Delay3/1
  Delay4/1 -> Integrator/2(validIn)
  Delay2/1 -> Integrator/1(dataIn)
  Delay1/1 -> Delay7/1
  Unit Delay Enabled Synchronous/1 -> Delay12/1
  Delay9/1 -> Delay6/1
  Delay3/1 -> Delay4/1
  Delay5/1 -> Gain1/1
  Gain1/1 -> Delay2/1
  Product/1 -> Delay5/1
  Math Function/1 -> Delay8/1
  Delay10/1 -> Extract Frequency/1(datain)
  Delay11/1 -> Extract Frequency/2(validIn)
  Integrator/1(IntegOut) -> Delay10/1
  Integrator/2(IntegValid) -> Delay11/1
  Extract Frequency/1(normFreqOut) -> normFreqEst/1
  dataIn/1 -> Delay1/1, Unit Delay Enabled Synchronous/1
  validIn/1 -> Unit Delay Enabled Synchronous/2, Delay9/1
  Delay12/1 -> Math Function/1

== system commhdlQPSKTxRx/Receiver/QPSK Rx/Frequency and Time Synchronizer/Coarse Frequency Compensator/Raise Power to 4 ==
  dataIn : Inport
  validIn : Inport  Port=2
  Delay{1..8,11..12} (10 alike) : Delay
  Delay10 : Delay  DelayLength=1
  Delay9 : Delay  DelayLength=1
  Product1 : Product  OutDataTypeStr=Inherit: Same as first input
  Product2 : Product  OutDataTypeStr=Inherit: Same as first input
  dataOut : Outport
  validOut : Outport  Port=2
  wires:
  Delay12/1 -> validOut/1
  Delay11/1 -> dataOut/1
  Delay10/1 -> Delay8/1
  Delay9/1 -> Delay6/1, Delay7/1
  Delay8/1 -> Delay12/1
  Delay7/1 -> Product2/2
  Delay6/1 -> Product2/1
  Delay5/1 -> Delay2/1
  Delay4/1 -> Product1/2
  Delay3/1 -> Product1/1
  validIn/1 -> Delay5/1
  Product2/1 -> Delay11/1
  Delay2/1 -> Delay10/1
  Product1/1 -> Delay1/1
  Delay1/1 -> Delay9/1
  dataIn/1 -> Delay4/1, Delay3/1

== system commhdlQPSKTxRx/Receiver/QPSK Rx/Frequency and Time Synchronizer/No HDL/Subsystem ==
  In1 : Inport
  Enable : EnablePort
  To Workspace : ToWorkspace  VariableName=simAfterCS  SampleTime=-1
      settings: Save2DSignal=2-D array (concatenate along first dimension)
  wires:
  In1/1 -> To Workspace/1

== system commhdlQPSKTxRx/Receiver/QPSK Rx/Frequency and Time Synchronizer/Packet Controller/End Generator ==
  validIn : Inport
  rst : Inport  Port=2
  Compare To Constant : simulink/Logic and Bit Operations/Compare To Constant  relop===  const=1120-1  OutDataTypeStr=boolean
  Delay6 : Delay  DelayLength=1
  HDL Counter : hdlsllib/Sources/HDL Counter  CountType=Count limited  CountInit=0  CountStep=1  CountMax=1120 -1  CountFromType=Initial value  CountFrom=0  CountResetPort=on  CountLoadPort=off  CountEnbPort=on  CountDirPort=off  CountHitOutputPort=off  CountDataType=Unsigned  CountWordLen=nextpow2(1120-1)  CountFracLen=0  CountSampTime=1
  Logical Operator1 : Logic  IconShape=distinctive  AllPortsSameDT=off  OutDataTypeStr=boolean
  endOut : Outport
  wires:
  Compare To Constant/1 -> Logical Operator1/1
  HDL Counter/1 -> Compare To Constant/1
  validIn/1 -> HDL Counter/2, Logical Operator1/2
  rst/1 -> HDL Counter/1
  Logical Operator1/1 -> Delay6/1
  Delay6/1 -> endOut/1

== system commhdlQPSKTxRx/Receiver/QPSK Rx/Frequency and Time Synchronizer/Phase Ambiguity Estimation and Correction/Average Estimates ==
  endIn : Inport
  estin : Inport  Port=2
  validIn : Inport  Port=3
  Add : Sum  Inputs=++|
  Data Type Conversion : DataTypeConversion  OutDataTypeStr=fixdt(1,16+8,13)  SaturateOnIntegerOverflow=off  RndMeth=Floor
  Data Type Conversion1 : DataTypeConversion  OutDataTypeStr=fixdt(1,16+8,13)  SaturateOnIntegerOverflow=off  RndMeth=Floor
  Data Type Conversion2 : DataTypeConversion  OutDataTypeStr=fixdt(1,16,14)  SaturateOnIntegerOverflow=off  RndMeth=Floor
  Delay{,1..3} (4 alike) : Delay  DelayLength=1
  Divide by 8 : DataTypeConversion  OutDataTypeStr=fixdt(1,24,13+log2(8))  ConvertRealWorld=Stored Integer (SI)  SaturateOnIntegerOverflow=off  RndMeth=Floor
  Unit Delay Enabled Synchronous : hdlsllib/Discrete/Unit Delay Enabled Synchronous  InitialCondition=0.0  SampleTime=-1
  Unit Delay Enabled Resettable Synchronous : hdlsllib/Discrete/Unit Delay Enabled Resettable Synchronous  InitialCondition=0.0  SampleTime=-1
  avgEst : Outport
  wires:
  validIn/1 -> Delay1/1
  estin/1 -> Delay/1
  Data Type Conversion/1 -> Add/2
  Add/1 -> Data Type Conversion1/1
  Unit Delay Enabled Resettable Synchronous/1 -> Add/1, Divide by 8/1
  Data Type Conversion1/1 -> Unit Delay Enabled Resettable Synchronous/1
  Delay/1 -> Data Type Conversion/1
  Delay1/1 -> Unit Delay Enabled Resettable Synchronous/2
  endIn/1 -> Delay2/1
  Delay2/1 -> Delay3/1, Unit Delay Enabled Synchronous/2
  Delay3/1 -> Unit Delay Enabled Resettable Synchronous/3
  Divide by 8/1 -> Unit Delay Enabled Synchronous/1
  Unit Delay Enabled Synchronous/1 -> Data Type Conversion2/1
  Data Type Conversion2/1 -> avgEst/1

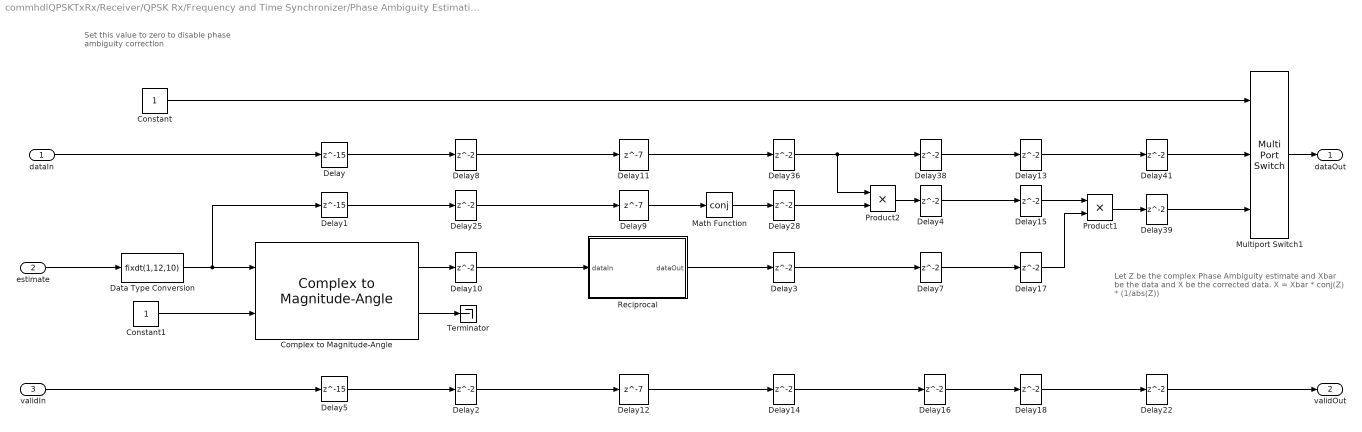
== system commhdlQPSKTxRx/Receiver/QPSK Rx/Frequency and Time Synchronizer/Phase Ambiguity Estimation and Correction/Phase Ambiguity Corrector ==
  note: Let Z be the complex Phase Ambiguity estimate and Xbar be the data and X be the corrected data.
      | X = Xbar * conj(Z) * (1/abs(Z))
  note: Set this value to zero to disable phase ambiguity correction
  dataIn : Inport
  estimate : Inport  Port=2
  validIn : Inport  Port=3
  Complex to Magnitude-Angle : dsphdlmathfun2/Complex to Magnitude-Angle  NumIterationsSource=Auto  NumIterations=10  OutputFormat=Magnitude  AngleFormat=Normalized  ScaleOutput=on  ScalingMethod=Shift-Add  SimulateUsing=Code generation
  Constant : Constant  OutDataTypeStr=boolean  SampleTime=-1
  Constant1 : Constant  OutMin=1  OutMax=1  OutDataTypeStr=boolean  SampleTime=-1
  Data Type Conversion : DataTypeConversion  OutDataTypeStr=fixdt(1,12,10)  SaturateOnIntegerOverflow=off  RndMeth=Floor
  Delay : Delay  DelayLength=15
  Delay1 : Delay  DelayLength=15
  Delay{2..4,7..8,10,13..18,22,25,28,36,38..39,41} (19 alike) : Delay  InitialCondition=0
  Delay11 : Delay  DelayLength=7  InitialCondition=0
  Delay12 : Delay  DelayLength=7  InitialCondition=0
  Delay5 : Delay  DelayLength=15
  Delay9 : Delay  DelayLength=7  InitialCondition=0
  Math Function : Math  Operator=conj  SignedPower=on  RndMeth=Zero
  Multiport Switch1 : MultiPortSwitch  DataPortOrder=Zero-based contiguous  Inputs=2  zeroidx=on  SaturateOnIntegerOverflow=off  InputSameDT=off
  Product1 : Product  OutDataTypeStr=Inherit: Same as first input
  Product2 : Product  OutDataTypeStr=Inherit: Same as first input
  Reciprocal : Subsystem  mask{WL=13, FL=10, outWL=26, Mapp=RAM - Based}
      mask prompts: WL "Input Word Length :"; FL "Input Fractional Length :"; outWL "Output Word Length :"; Mapp "Mapping Type:"
      mask init:
      | % Inverse for 18 bit numbers: partitioned into 3+15 bits. 2^3 LUTs with 2^15
      | % combinations will store a total of 2^18 combinations.
      | % As each LUT has 2^15 combinations the data type of output has a maximum
      | % limit of 32 bits (2^20 is a maximum number of bits an LUT can store)
      | 
      | % Non tunable Parameters
      | % FL = 16;
      | % outWL = 31;
      | % WL = 18;
      | % This Parameter is not given for mask
      | LUTAddrWL = WL - 1; % this will implement 2 LUTs
      | 
      | % validate Non tunable parameters
      | % condition for validation: 2^20 bits is the maximum number of bits an LUT can store
      | if LUTAddrWL >= 20   % As 2^20 is the limit
      |     error('invalid LUTAddrWL');
      | end
      | if outWL >= 2^(20-LUTAddrWL)  % 2^(20-LUTAddrWL) is the maximum outWL based on condition for validation
      |     error('invalid outWL')
      | end
      | 
      | % calculate number of LUTs required
      | muxSelectorWL = WL - LUTAddrWL;
      | nLUT = 2^muxSelectorWL;
      | 
      | % Generate all possible RWV inputs using WL and FL
      | allInputRangeSI = -2^(WL-1):2^(WL-1)-1;  % as a stored integer
      | allInputRWV = allInputRangeSI * 2^(-FL);
      | 
      | % define the function for all the RWV input
      | reciprocal = 1./allInputRWV;
      | 
      | % store the function output in LUT
      | allLUTAddr = (0:2^LUTAddrWL-1);
      | LUT = zeros(length(allLUTAddr),nLUT);
      | for i = 0:nLUT-1
      |     LUT(:,i+1) = reciprocal(i*2^LUTAddrWL+1:(i+1)*2^LUTAddrWL);
      | end
      | 
      | % quantize the function with outWL
      | NT = numerictype(fi(LUT(abs(LUT) ~= inf),1,outWL)); % inf and -inf will be quantized with max and min values with NT data type
      | if NT.WordLength < NT. FractionLength
      |     NT.FractionLength = NT.WordLength
      | end
      | LUT = fi(LUT,NT);
      | 
      | paths = find_system([gcb '/Function Impl'],'BlockType','Delay');
      | 
      | for i = 1:length(paths)
      |     if Mapp == 1
      |         hdlset_param(paths{i},'ResetType','default');
      |     else
      |         hdlset_param(paths{i},'ResetType','none');
      |     end
      | end
      mask TypeOptions Mapp: LUT - Based | RAM - Based
      mask DialogControl DescGroupVar Prompt: LUT - Based function
      mask DialogControl DescTextVar Prompt: This block is implemented for complex reciprocal
      mask Display: disp(['Reciprocal\n' get_param(gcb,'Mapp') '\nLatency = 7'])
  Terminator : Terminator
  dataOut : Outport
  validOut : Outport  Port=2
  wires:
  Delay3/1 -> Delay7/1
  Delay18/1 -> Delay22/1
  Delay17/1 -> Product1/2
  Delay15/1 -> Product1/1
  Delay13/1 -> Delay41/1
  Delay10/1 -> Reciprocal/1(dataIn)
  Delay12/1 -> Delay14/1
  Delay11/1 -> Delay36/1
  Delay9/1 -> Math Function/1
  Delay4/1 -> Delay15/1
  Delay41/1 -> Multiport Switch1/2
  Delay8/1 -> Delay11/1
  Delay/1 -> Delay8/1
  dataIn/1 -> Delay/1
  validIn/1 -> Delay5/1
  Delay5/1 -> Delay2/1
  Delay2/1 -> Delay12/1
  Delay14/1 -> Delay16/1
  Product2/1 -> Delay4/1
  Multiport Switch1/1 -> dataOut/1
  Delay22/1 -> validOut/1
  Constant/1 -> Multiport Switch1/1
  Delay16/1 -> Delay18/1
  Delay28/1 -> Product2/2
  Math Function/1 -> Delay28/1
  Delay25/1 -> Delay9/1
  Delay1/1 -> Delay25/1
  Delay36/1 -> Product2/1, Delay38/1
  Delay38/1 -> Delay13/1
  estimate/1 -> Data Type Conversion/1
  Reciprocal/1(dataOut) -> Delay3/1
  Product1/1 -> Delay39/1
  Constant1/1 -> Complex to Magnitude-Angle/2
  Complex to Magnitude-Angle/1 -> Delay10/1
  Complex to Magnitude-Angle/2 -> Terminator/1
  Delay39/1 -> Multiport Switch1/3
  Delay7/1 -> Delay17/1
  Data Type Conversion/1 -> Delay1/1, Complex to Magnitude-Angle/1
